simulink subsystem "Gyro_Angles_sub"  (R2023b)
settings: Solver=VariableStepAuto  StartTime=0.0  StopTime=10.0  RelTol=1e-3
undefined symbols (not defined in the file): Gyro_Calibration_Default, Gyro_Calibration_Reset_Flag, RobotMaxV_GyroReset
libraries: simulink x3, simulink_extras x3, Controls_Components_lib x2
settings Model: Creator=ander  LastModifiedBy=ander

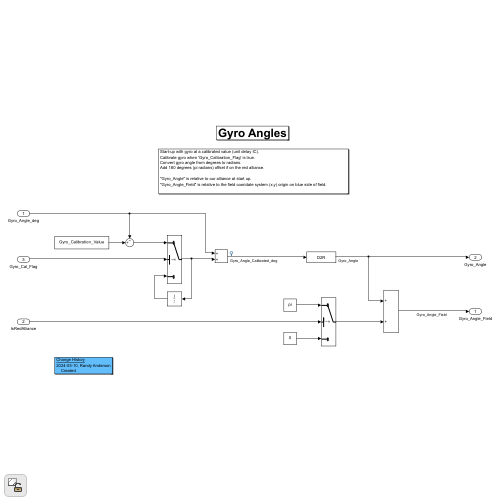
[thumbnail: Simulink's stored preview of the top-level diagram]
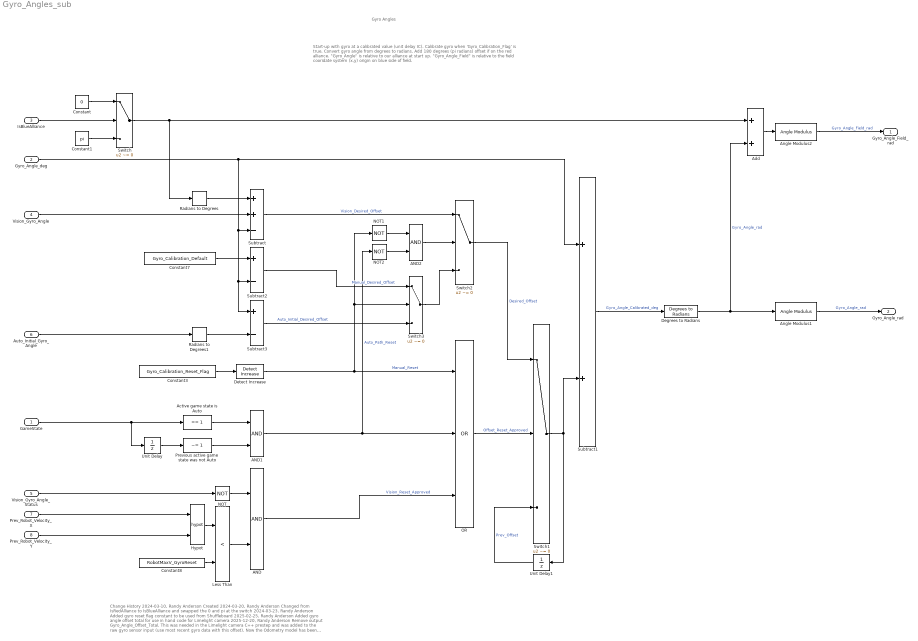
== system Gyro_Angles_sub ==
  note: Gyro Angles
  note: Start-up with gyro at a calibrated value (unit delay IC).
      | Calibrate gyro when 'Gyro_Calibration_Flag' is true.
      | Convert gyro angle from degrees to radians.
      | Add 180 degrees (pi radians) offset if on the red alliance.
      |
      | "Gyro_Angle" is relative to our alliance at start up.
      | "Gyro_Angle_Field" is relative to the field cooridate system (x,y) origin on blue side of field.
  note: Change History
      | 2024-03-10, Randy Anderson
      | Created
      | 2024-03-20, Randy Anderson
      | Changed from IsRedAlliance to IsBlueAlliance and swapped the 0 and pi at the switch
      | 2024-03-23, Randy Anderson
      | Added gyro reset flag constant to be used from Shuffleboard
      | 2025-02-25, Randy Anderson
      | Added gyro angle offset total for use in hand code for Limelight camera
      | 2025-12-20, Randy Anderson
      | Remove output Gyro_Angle_Offset_Total. This was needed in the Limelight camera C++ prestep and was added to the raw gyro
      | sensor input (use most recent gyro data with this offset). Now the Odometry model has been split out and runs before the Limelight
      | camera prestep, so we can instead use Gyro_Angle_Field_rad (with conversion to degrees in C++) which already includes the offsets.
      | 2026-2-28, Wyatt Kromer & Anirudh
      | Added capability for limlight input to update our gyro offset as long as we're recieving a valid target and the robot is going slow enough.
      | 2026-03-08, Randy Anderson & Wyatt Kromer
      | Added reset to the initial value at start of autonomous routine. Pull value from external interface which comes from Autos.
  GameState : Inport
  Gyro_Angle_deg : Inport  Port=2
  IsBlueAlliance : Inport  Port=3
  Vision_Gyro_Angle : Inport  Port=4
  Vision_Gyro_Angle_Status : Inport  Port=5
  Auto_Initial_Gyro_Angle : Inport  Port=6
  Prev_Robot_Velocity_X : Inport  Port=7
  Prev_Robot_Velocity_Y : Inport  Port=8
  AND : Logic  AllPortsSameDT=off  OutDataTypeStr=boolean
  AND1 : Logic  AllPortsSameDT=off  OutDataTypeStr=boolean
  AND2 : Logic  AllPortsSameDT=off  OutDataTypeStr=boolean
  Active game state is Auto : simulink/Logic and Bit Operations/Compare To Constant  relop===  const=1  OutDataTypeStr=boolean
  Add : Sum
  Angle Modulus1 : Controls_Components_lib/Angle Modulus  SystemSampleTime=-1  VariantActivationTime=update diagram  AllowFlexibleInterface=on  Latency=0  AutoFrameSizeCalculation=off
  Angle Modulus2 : Controls_Components_lib/Angle Modulus  SystemSampleTime=-1  VariantActivationTime=update diagram  AllowFlexibleInterface=on  Latency=0  AutoFrameSizeCalculation=off
  Constant : Constant  Value=0
  Constant1 : Constant  Value=pi
  Constant3 : Constant  Value=Gyro_Calibration_Reset_Flag
  Constant7 : Constant  Value=Gyro_Calibration_Default  OutDataTypeStr=double
  Constant8 : Constant  Value=RobotMaxV_GyroReset
  Degrees to Radians : simulink_extras/Transformations/Degrees to Radians
  Detect Increase : simulink/Logic and Bit Operations/Detect Increase  vinit=0.0  OutDataTypeStr=boolean
  Hypot : Math  Operator=hypot
  Less Than : RelationalOperator  Operator=<  OutDataTypeStr=boolean  RndMeth=Simplest  InputSameDT=off
  NOT : Logic  Operator=NOT  AllPortsSameDT=off  OutDataTypeStr=boolean
  NOT1 : Logic  Operator=NOT  AllPortsSameDT=off  OutDataTypeStr=boolean
  NOT2 : Logic  Operator=NOT  AllPortsSameDT=off  OutDataTypeStr=boolean
  OR : Logic  Operator=OR  Inputs=3  AllPortsSameDT=off  OutDataTypeStr=boolean
  Previous active game state was not Auto : simulink/Logic and Bit Operations/Compare To Constant  relop=~=  const=1  OutDataTypeStr=boolean
  Radians to Degrees : simulink_extras/Transformations/Radians to Degrees
  Radians to Degrees1 : simulink_extras/Transformations/Radians to Degrees
  Subtract : Sum  Inputs=++-
  Subtract1 : Sum
  Subtract2 : Sum  Inputs=+-
  Subtract3 : Sum  Inputs=+-
  Switch{,1..3} (4 alike) : Switch  Criteria=u2 ~= 0  SaturateOnIntegerOverflow=off  InputSameDT=off
  Unit Delay : UnitDelay  SampleTime=-1  HasFrameUpgradeWarning=on
  Unit Delay1 : UnitDelay  InitialCondition=Gyro_Calibration_Default  SampleTime=-1  HasFrameUpgradeWarning=on
  Gyro_Angle_Field_rad : Outport
  Gyro_Angle_rad : Outport  Port=2
  wires:
  Add/1 -> Angle Modulus2/1
  Degrees to Radians/1 -> Angle Modulus1/1, Add/2  "Gyro_Angle_rad"
  IsBlueAlliance/1 -> Switch/2
  Constant/1 -> Switch/1
  Constant1/1 -> Switch/3
  Unit Delay1/1 -> Switch1/3  "Prev_Offset"
  Switch1/1 -> Unit Delay1/1, Subtract1/2
  Switch2/1 -> Switch1/1  "Desired_Offset"
  Subtract1/1 -> Degrees to Radians/1  "Gyro_Angle_Calibrated_deg"
  Gyro_Angle_deg/1 -> Subtract2/2, Subtract3/1, Subtract/3, Subtract1/1
  Constant3/1 -> Detect Increase/1
  OR/1 -> Switch1/2  "Offset_Reset_Approved"
  Vision_Gyro_Angle_Status/1 -> NOT/1
  Vision_Gyro_Angle/1 -> Subtract/2
  Prev_Robot_Velocity_X/1 -> Hypot/1
  Prev_Robot_Velocity_Y/1 -> Hypot/2
  Hypot/1 -> Less Than/1
  Less Than/1 -> AND/2
  Constant8/1 -> Less Than/2
  NOT/1 -> AND/1
  Subtract/1 -> Switch2/1  "Vision_Desired_Offset"
  Detect Increase/1 -> NOT1/1, Switch3/2, OR/1  "Manual_Reset"
  Angle Modulus2/1 -> Gyro_Angle_Field_rad/1  "Gyro_Angle_Field_rad"
  Angle Modulus1/1 -> Gyro_Angle_rad/1  "Gyro_Angle_rad"
  Switch/1 -> Radians to Degrees/1, Add/1
  Constant7/1 -> Subtract2/1
  GameState/1 -> Active game state is Auto/1, Unit Delay/1
  Unit Delay/1 -> Previous active game state was not Auto/1
  Previous active game state was not Auto/1 -> AND1/2
  Active game state is Auto/1 -> AND1/1
  AND1/1 -> OR/2, NOT2/1  "Auto_Path_Reset"
  Auto_Initial_Gyro_Angle/1 -> Radians to Degrees1/1
  Radians to Degrees1/1 -> Subtract3/2
  NOT1/1 -> AND2/1
  NOT2/1 -> AND2/2
  AND2/1 -> Switch2/2
  Switch3/1 -> Switch2/3
  Subtract2/1 -> Switch3/1  "Manual_Desired_Offset"
  Subtract3/1 -> Switch3/3  "Auto_Initial_Desired_Offset"
  AND/1 -> OR/3  "Vision_Reset_Approved"
  Radians to Degrees/1 -> Subtract/1
